simulink model "UART"  (Simulink 7.1)
settings: Solver=FixedStepDiscrete  StartTime=0.0  StopTime=10.0  FixedStep=0.001  RelTol=1e-3
libraries: dsPICdrivers x5
settings Model: Creator=ARGULIO  LastModifiedBy=ARGULIO
settings OptimizationCC: OptimizeModelRefInitCode=on  LifeSpan=1
settings HardwareCC: ProdBitPerInt=16  ProdEndianess=LittleEndian  ProdWordSize=16  ProdHWDeviceType=16-bit Generic
settings RTWCC: SystemTargetFile=dspic.tlc  GenerateMakefile=off  TemplateMakefile=dspic_pic30_gcc.tmf  PostCodeGenCommand=dsPIC_Compile()  Description=Embedded Target for Microchip dsPIC (real-time)  ProcessScript=dspic_make_rtw_hook
settings CodeAppCC: IgnoreCustomStorageClasses=off
settings STFCustomTargetCC: ModelReferenceCompliant=off  IncludeMdlTerminateFcn=off  CombineOutputUpdateFcns=on  SuppressErrorStatus=on  ERTCustomFileBanners=on  SupportContinuousTime=off  SupportNonInlinedSFcns=off  SystemTargetFile=dspic.tlc
settings ERTTargetCC: ModelReferenceCompliant=off  CompOptLevelCompliant=off  IncludeMdlTerminateFcn=off  SuppressErrorStatus=on  ERTFirstTimeCompliant=off  ModelStepFunctionPrototypeControlCompliant=off  ExtModeMexFile=noextcomm  InlinedParameterPlacement=NonHierarchical  ERTSrcFileBannerTemplate=dsPIC_code_template.cgt  ERTHdrFileBannerTemplate=dsPIC_code_template.cgt  ERTDataSrcFileTemplate=dsPIC_code_template.cgt  ERTDataHdrFileTemplate=dsPIC_code_template.cgt  ERTCustomFileTemplate=dsPIC_main.tlc
settings CustomProperty: DataType=string  Value=C:\PROGRA~1\MATLAB\R2008a\bin\win32\gmake

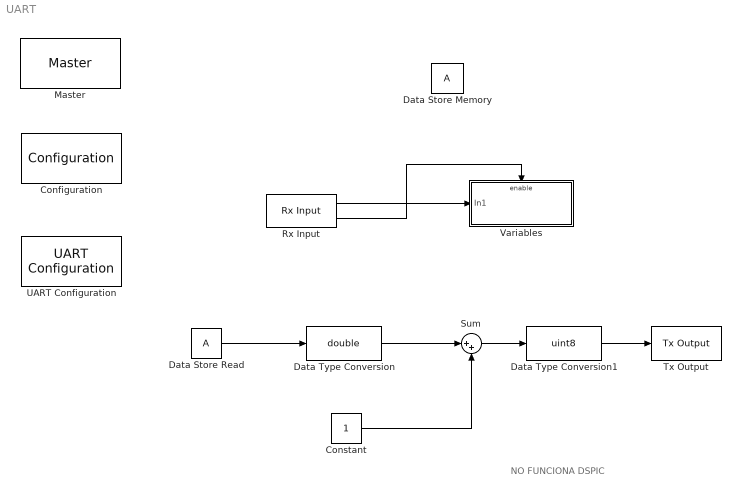
== system UART ==
  note: NO FUNCIONA DSPIC
  Configuration : dsPICdrivers/Configuration  SystemSampleTime=-1  double64=off
  Constant : Constant  OutDataType=sfix(16)  OutScaling=2^0
  Data Store Memory : DataStoreMemory  DataStoreName=A  ReadBeforeWriteMsg=warning  WriteAfterWriteMsg=warning  WriteAfterReadMsg=warning  InitialValue=255  DataType=uint8  OutDataType=sfix(16)  OutScaling=2^0  OutDataTypeStr=uint8
  Data Store Read : DataStoreRead  DataStoreName=A  SampleTime=-1
  Data Type Conversion : DataTypeConversion  OutDataTypeMode=double  OutDataType=sfix(16)  OutScaling=2^0  OutDataTypeStr=double
  Data Type Conversion1 : DataTypeConversion  OutDataTypeMode=uint8  OutDataType=sfix(16)  OutScaling=2^0  OutDataTypeStr=uint8
  Master : dsPICdrivers/Master  Tag=dsPIC_MASTER  Priority=1  TimeStepType=Timer1  picType=33fJ256GP710  fcy=2500000  Quartz_33f=5e6  PLLActive_33f=off  fcyDesired_33f=0  tmr1="[1  2499  0]"  tmr1Info="Time Step : 0.001  ;   Error : 0%  PR1=2499"  tmr2345="[0  0  0  0  0  0  0  0]"  tmr2345cfg=[-1 -1 -1 -1 -1 -1 -1 -1]  IOautoConf=on  typePort="[ 0  0  0  0  0  0  0  0  0  0  0  0  0  0  0  0  0  0  0  0  0  0  0  0  0  0  0  0  0  0  0  0  0  0  0  0  0  0  0  0  0  0  0  0  0  0  0  0  0  0  0  0  0  0  0  0  0  0  0  0  0  0  0  0  0  0  0  0  0  0  0  0  0  0  0  0  0  0  0  0  0  0  4  5  0  0  0  0  0  0  0  0  0  0  0  0  0  0  0  0  0  0  0  0  0  0  0  0  0  0  0  0 ]"  TRIS="[ 65535  65535  65535  65535  65535  65535  65535 ]"  ADPCFG=0  MasterBusyPort=None  MasterOverloadPort=None  FOSC=Quartz (XT - HS)  ClockSwitchMonitor=Both disabled  TempProtection_33f=TEMP_ON  FPBOR=<empty>  PWRT=disable  MCLR=<empty>  PowerSave=off  OverrideFcy=off  NewFcy=1e6  PR2345="[65535  65535  65535  65535  65535  65535  65535  65535]"
  Rx Input : dsPICdrivers/Serial PORT/Rx Input  Tag=dsPIC_RX  Priority=5  UART=1  SampleTime=-1  BlockingFctChk=off  OutputDefault=0  IsPresentFlagChk=on
  Sum : Sum  Inputs=|++  OutDataType=sfix(16)  OutScaling=2^0
  Tx Output : dsPICdrivers/Serial PORT/Tx Output  Tag=dsPIC_TX  Priority=5  UART=1  OrderingInOutPopup=None
  UART Configuration : dsPICdrivers/Serial PORT/UART Configuration  Tag=dsPIC_config_UART  Priority=2  UART=1  proposed_BAUD=300  ALT_TX_RX=on  InterruptTxWhen=When Transmit Buffer is empty  TXInterruptPri=2  TxBufferSize=32  TXEN=on  InterruptRxWhen=When a character is received  RXInterruptPri=1  RxBufferSize=32  BAUD=300  UxBRG=520  Info="UxBRG = 520   ||  Real Baud : 300   ||  % error : -0.03199  ||  max 0.02999 Bytes / Step"  RealBaud=0
  Variables : Subsystem  TreatAsAtomicUnit=on
  wires:
  Rx Input/1 -> Variables/1(In1)
  Rx Input/2 -> Variables/Enable
  Data Store Read/1 -> Data Type Conversion/1
  Data Type Conversion/1 -> Sum/1
  Sum/1 -> Data Type Conversion1/1
  Constant/1 -> Sum/2
  Data Type Conversion1/1 -> Tx Output/1

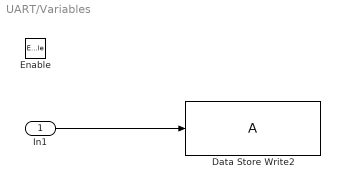
== system UART/Variables ==
  In1 : Inport  OutDataType=sfix(16)  OutScaling=2^0
  Enable : EnablePort
  Data Store Write2 : DataStoreWrite  DataStoreName=A  SampleTime=-1
  wires:
  In1/1 -> Data Store Write2/1
